simulink model "MMC_phase_discentralized_HAAS_20260927"  (R2024b)
settings: Solver=FixedStepDiscrete  StartTime=t_init_sim  StopTime=sim_time  FixedStep=Ts  RelTol=1e-3
values from neighbouring files (symbols this model uses):
  a = 1    [script_MMC_phase_hackathon_NLM_discentralized_HAAS_20260927.m]
  C1low1_active = 1    [script_MMC_phase_hackathon_NLM_discentralized_HAAS_20260927.m]
  C2low1_active = 1    [script_MMC_phase_hackathon_NLM_discentralized_HAAS_20260927.m]
  C_bus = 4400e-6    (= 0.0044)    [script_MMC_phase_hackathon_NLM_discentralized_HAAS_20260927.m]
  C_M_extra = C_m-twist_high_side_C    [script_MMC_phase_hackathon_NLM_discentralized_HAAS_20260927.m]
  duty_cycle = 1.0    (= 1)    [script_MMC_phase_hackathon_NLM_discentralized_HAAS_20260927.m]
  f0 = 50    [script_MMC_phase_hackathon_NLM_discentralized_HAAS_20260927.m]
  feeder_current_lower_rate_limit = -10    [script_MMC_phase_hackathon_NLM_discentralized_HAAS_20260927.m]    (also in twist_parameters.m = -500)
  feeder_current_tab = [0.328 0.217 0.162 0.132 0.109 0.094 0.083 0.075 0.068 0.062 0.058 0.054 ... (42 elements, 14x3)]    [feeder_current.mat]
  feeder_current_upper_rate_limit = 0.386/(20e-3)    (= 19.3)    [twist_parameters.m]
  is6VExternallySupplied = true    [script_MMC_phase_hackathon_NLM_discentralized_HAAS_20260927.m]
  isFeederJumperOpen = true    [script_MMC_phase_hackathon_NLM_discentralized_HAAS_20260927.m]
  L_arm = 30e-3    (= 0.03)    [script_MMC_phase_hackathon_NLM_discentralized_HAAS_20260927.m]
  m = 1    [script_MMC_phase_hackathon_NLM_discentralized_HAAS_20260927.m]
  N = 5    [script_MMC_phase_hackathon_NLM_discentralized_HAAS_20260927.m]
  power_losses = false    [script_MMC_phase_hackathon_NLM_discentralized_HAAS_20260927.m]
  R = 15    [script_MMC_phase_hackathon_NLM_discentralized_HAAS_20260927.m]
  R_arm = 0.2    [script_MMC_phase_hackathon_NLM_discentralized_HAAS_20260927.m]
  source_V = 0    [script_MMC_phase_hackathon_NLM_discentralized_HAAS_20260927.m]
  Tcom_sample = round(Tcom / Ts)    [script_MMC_phase_hackathon_NLM_discentralized_HAAS_20260927.m]
  time_charge = 0.1    [script_MMC_phase_hackathon_NLM_discentralized_HAAS_20260927.m]
  time_decharge = 1.5    [script_MMC_phase_hackathon_NLM_discentralized_HAAS_20260927.m]
  Ts = 1e-6    (= 1e-06)    [script_MMC_phase_hackathon_NLM_discentralized_HAAS_20260927.m]
  twist_data_acquisition_delay = 50e-9    (= 5e-08)    [script_MMC_phase_hackathon_NLM_discentralized_HAAS_20260927.m]    (also in twist_parameters.m)
  twist_data_sampling_period = 1/twist_freq_data_sampling    (= 5e-05)    [script_MMC_phase_hackathon_NLM_discentralized_HAAS_20260927.m]    (also in twist_parameters.m)
  twist_dead_time = 200e-9    (= 2e-07)    [twist_parameters.m]
  twist_freq_switching = 200e3    (= 200000)    [twist_parameters.m]
  twist_high_side_adc_R = 1/(1/2e6 + 1/2e6 + 1/(330e3+5.6e3))    (= 251272.836178)    [twist_parameters.m]
  twist_high_side_C = 33e-6*4 + 4.7e-6*12    (= 0.0001884)    [twist_parameters.m]
  twist_high_side_feeder_R = 47e3+4.7e3    (= 51700)    [twist_parameters.m]
  twist_high_side_rC = 0.1    [twist_parameters.m]
  twist_low_side_adc_R = 150e3+470    (= 150470)    [twist_parameters.m]
  twist_low_side_C_ceramic = 3*4.7e-6    (= 1.41e-05)    [twist_parameters.m]
  twist_low_side_C_electrolytic = 47e-6    (= 4.7e-05)    [twist_parameters.m]
  twist_low_side_L = 33e-6    (= 3.3e-05)    [twist_parameters.m]
  twist_low_side_rC = 700e-3    (= 0.7)    [twist_parameters.m]
  twist_low_side_rL = 20e-3    (= 0.02)    [twist_parameters.m]
  twist_R_VCC = (tau_VCC/twist_high_side_C  - twist_high_side_rC)/(1-(tau_VCC/twist_high_side_C - twist_high_side_rC)/R_parallel)    (= 1110.74997822)    [twist_parameters.m]
  VDC = 48    [script_MMC_phase_hackathon_NLM_discentralized_HAAS_20260927.m]
undefined symbols (not defined in the file or in its folder): C_SM, feeder_current, gcbh, sps_rtmsupport, twist_low_side_lC
libraries: spsSeriesRLCBranchLib x135, spsTriangleGeneratorLib x60, spsMosfetLib x60, spsCurrentMeasurementLib x43, spsVoltageMeasurementLib x35, spsControlledCurrentSourceLib x30, spsDiodeLib x22, spsIdealSwitchLib x20, spsControlledVoltageSourceLib x1, spsGroundLib x1, spspowerguiLib x1
(part 18 of 22)

== system MMC_phase_discentralized_HAAS_20260927/ /Subsystem/Subsystem1/Hardware M5/HRTimA_1/PWM Generator (2-Level)/Sampling/Unsync Natural/Unsync_NaturalSampling ==
  Uref : Inport  Interpolate=off
  Triangle Generator : spsTriangleGeneratorLib/Triangle Generator  Freq=sps.Fc  Phase=sps.Pc  Ts=Ts
  Uref* : Outport  VectorParamsAs1DForOutWhenUnconnected=off
  Cr : Outport  Port=2  VectorParamsAs1DForOutWhenUnconnected=off
  wires:
  Triangle Generator/1 -> Cr/1
  Uref/1 -> Uref*/1

== system MMC_phase_discentralized_HAAS_20260927/ /Subsystem/Subsystem1/Hardware M5/HRTimA_1/PWM Generator (2-Level)/Sampling/Unsync Symmetrical/Unsync_SymmetricalSampling ==
  Uref : Inport  Interpolate=off
  Triangle Generator : spsTriangleGeneratorLib/Triangle Generator  Freq=sps.Fc  Phase=sps.Pc  Ts=Ts
  Zero-Order Hold : ZeroOrderHold  SampleTime=sps.SampleTimeZOH_SymSampling
  Uref* : Outport  VectorParamsAs1DForOutWhenUnconnected=off
  Cr : Outport  Port=2  VectorParamsAs1DForOutWhenUnconnected=off
  wires:
  Triangle Generator/1 -> Cr/1
  Uref/1 -> Zero-Order Hold/1
  Zero-Order Hold/1 -> Uref*/1

== system MMC_phase_discentralized_HAAS_20260927/ /Subsystem/Subsystem1/Hardware M5/HRTimA_2/PWM Generator (2-Level)/Sampling/Sync Asymmetrical/Sample & Hold ==
  In : Inport
  Enable : EnablePort
  Out : Outport  VectorParamsAs1DForOutWhenUnconnected=off
  wires:
  In/1 -> Out/1

== system MMC_phase_discentralized_HAAS_20260927/ /Subsystem/Subsystem1/Hardware M5/HRTimA_2/PWM Generator (2-Level)/Sampling/Sync Natural/Sync_NaturalSampling ==
  Uref : Inport  Interpolate=off
  wt : Inport  Port=2  Interpolate=off
  Gain1 : Gain  Gain=2/pi  SaturateOnIntegerOverflow=on  OutDataTypeStr=Inherit: Same as input  ParamDataTypeStr=Inherit: Same as input
  Gain4 : Gain  Gain=nF  SaturateOnIntegerOverflow=on  OutDataTypeStr=Inherit: Same as input  ParamDataTypeStr=Inherit: Same as input
  Trigonometric Function : Trigonometry  Operator=asin
  Trigonometric Function3 : Trigonometry
  Uref* : Outport  VectorParamsAs1DForOutWhenUnconnected=off
  Cr : Outport  Port=2  VectorParamsAs1DForOutWhenUnconnected=off
  wires:
  wt/1 -> Gain4/1
  Gain1/1 -> Cr/1
  Trigonometric Function/1 -> Gain1/1
  Trigonometric Function3/1 -> Trigonometric Function/1
  Gain4/1 -> Trigonometric Function3/1
  Uref/1 -> Uref*/1

== system MMC_phase_discentralized_HAAS_20260927/ /Subsystem/Subsystem1/Hardware M5/HRTimA_2/PWM Generator (2-Level)/Sampling/Sync Symmetrical/Sync_SymmetricalSampling ==
  Uref : Inport  Interpolate=off
  wt : Inport  Port=2  Interpolate=off
  Add : Sum
  Constant3 : Constant
  Gain1 : Gain  Gain=2/pi  SaturateOnIntegerOverflow=on  OutDataTypeStr=Inherit: Same as input  ParamDataTypeStr=Inherit: Same as input
  Gain4 : Gain  Gain=nF  SaturateOnIntegerOverflow=on  OutDataTypeStr=Inherit: Same as input  ParamDataTypeStr=Inherit: Same as input
  Hit Crossing : HitCross  HitCrossingOffset=1e-9  HitCrossingDirection=falling
  Sample & Hold : Subsystem
  Trigonometric Function : Trigonometry  Operator=asin
  Trigonometric Function3 : Trigonometry
  Uref* : Outport  VectorParamsAs1DForOutWhenUnconnected=off
  Cr : Outport  Port=2  VectorParamsAs1DForOutWhenUnconnected=off
  wires:
  wt/1 -> Gain4/1
  Gain1/1 -> Cr/1, Add/1
  Trigonometric Function/1 -> Gain1/1
  Trigonometric Function3/1 -> Trigonometric Function/1
  Gain4/1 -> Trigonometric Function3/1
  Add/1 -> Hit Crossing/1
  Constant3/1 -> Add/2
  Hit Crossing/1 -> Sample & Hold/Enable
  Uref/1 -> Sample & Hold/1(In)
  Sample & Hold/1(Out) -> Uref*/1

== system MMC_phase_discentralized_HAAS_20260927/ /Subsystem/Subsystem1/Hardware M5/HRTimA_2/PWM Generator (2-Level)/Sampling/Unsync Asymmetrical/Unsync_AsymmetricalSampling ==
  Uref : Inport  Interpolate=off
  Triangle Generator : spsTriangleGeneratorLib/Triangle Generator  Freq=sps.Fc  Phase=sps.Pc  Ts=Ts
  Zero-Order Hold : ZeroOrderHold  SampleTime=sps.SampleTimeZOH_AsymSampling
  Uref* : Outport  VectorParamsAs1DForOutWhenUnconnected=off
  Cr : Outport  Port=2  VectorParamsAs1DForOutWhenUnconnected=off
  wires:
  Triangle Generator/1 -> Cr/1
  Uref/1 -> Zero-Order Hold/1
  Zero-Order Hold/1 -> Uref*/1

== system MMC_phase_discentralized_HAAS_20260927/ /Subsystem/Subsystem1/Hardware M5/HRTimA_2/PWM Generator (2-Level)/Sampling/Unsync Natural/Unsync_NaturalSampling ==
  Uref : Inport  Interpolate=off
  Triangle Generator : spsTriangleGeneratorLib/Triangle Generator  Freq=sps.Fc  Phase=sps.Pc  Ts=Ts
  Uref* : Outport  VectorParamsAs1DForOutWhenUnconnected=off
  Cr : Outport  Port=2  VectorParamsAs1DForOutWhenUnconnected=off
  wires:
  Triangle Generator/1 -> Cr/1
  Uref/1 -> Uref*/1

== system MMC_phase_discentralized_HAAS_20260927/ /Subsystem/Subsystem1/Hardware M5/HRTimA_2/PWM Generator (2-Level)/Sampling/Unsync Symmetrical/Unsync_SymmetricalSampling ==
  Uref : Inport  Interpolate=off
  Triangle Generator : spsTriangleGeneratorLib/Triangle Generator  Freq=sps.Fc  Phase=sps.Pc  Ts=Ts
  Zero-Order Hold : ZeroOrderHold  SampleTime=sps.SampleTimeZOH_SymSampling
  Uref* : Outport  VectorParamsAs1DForOutWhenUnconnected=off
  Cr : Outport  Port=2  VectorParamsAs1DForOutWhenUnconnected=off
  wires:
  Triangle Generator/1 -> Cr/1
  Uref/1 -> Zero-Order Hold/1
  Zero-Order Hold/1 -> Uref*/1

== system MMC_phase_discentralized_HAAS_20260927/ /Subsystem/Subsystem/Hardware M1/HRTimA_1/PWM Generator (2-Level)/Sampling/Sync Symmetrical/Sync_SymmetricalSampling/Sample & Hold ==
  In : Inport
  Enable : EnablePort
  Out : Outport  VectorParamsAs1DForOutWhenUnconnected=off
  wires:
  In/1 -> Out/1

== system MMC_phase_discentralized_HAAS_20260927/ /Subsystem/Subsystem/Hardware M1/HRTimA_2/PWM Generator (2-Level)/Sampling/Sync Symmetrical/Sync_SymmetricalSampling/Sample & Hold ==
  In : Inport
  Enable : EnablePort
  Out : Outport  VectorParamsAs1DForOutWhenUnconnected=off
  wires:
  In/1 -> Out/1

== system MMC_phase_discentralized_HAAS_20260927/ /Subsystem/Subsystem/Hardware M2/HRTimA_1/PWM Generator (2-Level)/Sampling/Sync Symmetrical/Sync_SymmetricalSampling/Sample & Hold ==
  In : Inport
  Enable : EnablePort
  Out : Outport  VectorParamsAs1DForOutWhenUnconnected=off
  wires:
  In/1 -> Out/1

== system MMC_phase_discentralized_HAAS_20260927/ /Subsystem/Subsystem/Hardware M2/HRTimA_2/PWM Generator (2-Level)/Sampling/Sync Symmetrical/Sync_SymmetricalSampling/Sample & Hold ==
  In : Inport
  Enable : EnablePort
  Out : Outport  VectorParamsAs1DForOutWhenUnconnected=off
  wires:
  In/1 -> Out/1

== system MMC_phase_discentralized_HAAS_20260927/ /Subsystem/Subsystem/Hardware M3/HRTimA_1/PWM Generator (2-Level)/Sampling/Sync Symmetrical/Sync_SymmetricalSampling/Sample & Hold ==
  In : Inport
  Enable : EnablePort
  Out : Outport  VectorParamsAs1DForOutWhenUnconnected=off
  wires:
  In/1 -> Out/1

== system MMC_phase_discentralized_HAAS_20260927/ /Subsystem/Subsystem/Hardware M3/HRTimA_2/PWM Generator (2-Level)/Sampling/Sync Symmetrical/Sync_SymmetricalSampling/Sample & Hold ==
  In : Inport
  Enable : EnablePort
  Out : Outport  VectorParamsAs1DForOutWhenUnconnected=off
  wires:
  In/1 -> Out/1

== system MMC_phase_discentralized_HAAS_20260927/ /Subsystem/Subsystem/Hardware M4/HRTimA_1/PWM Generator (2-Level)/Sampling/Sync Symmetrical/Sync_SymmetricalSampling/Sample & Hold ==
  In : Inport
  Enable : EnablePort
  Out : Outport  VectorParamsAs1DForOutWhenUnconnected=off
  wires:
  In/1 -> Out/1

== system MMC_phase_discentralized_HAAS_20260927/ /Subsystem/Subsystem/Hardware M4/HRTimA_2/PWM Generator (2-Level)/Sampling/Sync Symmetrical/Sync_SymmetricalSampling/Sample & Hold ==
  In : Inport
  Enable : EnablePort
  Out : Outport  VectorParamsAs1DForOutWhenUnconnected=off
  wires:
  In/1 -> Out/1

== system MMC_phase_discentralized_HAAS_20260927/ /Subsystem/Subsystem/Hardware M5/HRTimA_1/PWM Generator (2-Level)/Sampling/Sync Symmetrical/Sync_SymmetricalSampling/Sample & Hold ==
  In : Inport
  Enable : EnablePort
  Out : Outport  VectorParamsAs1DForOutWhenUnconnected=off
  wires:
  In/1 -> Out/1

== system MMC_phase_discentralized_HAAS_20260927/ /Subsystem/Subsystem/Hardware M5/HRTimA_2/PWM Generator (2-Level)/Sampling/Sync Symmetrical/Sync_SymmetricalSampling/Sample & Hold ==
  In : Inport
  Enable : EnablePort
  Out : Outport  VectorParamsAs1DForOutWhenUnconnected=off
  wires:
  In/1 -> Out/1

== system MMC_phase_discentralized_HAAS_20260927/ /Subsystem/Subsystem1/Hardware M1/HRTimA_1/PWM Generator (2-Level)/Sampling/Sync Symmetrical/Sync_SymmetricalSampling/Sample & Hold ==
  In : Inport
  Enable : EnablePort
  Out : Outport  VectorParamsAs1DForOutWhenUnconnected=off
  wires:
  In/1 -> Out/1

== system MMC_phase_discentralized_HAAS_20260927/ /Subsystem/Subsystem1/Hardware M1/HRTimA_2/PWM Generator (2-Level)/Sampling/Sync Symmetrical/Sync_SymmetricalSampling/Sample & Hold ==
  In : Inport
  Enable : EnablePort
  Out : Outport  VectorParamsAs1DForOutWhenUnconnected=off
  wires:
  In/1 -> Out/1

== system MMC_phase_discentralized_HAAS_20260927/ /Subsystem/Subsystem1/Hardware M2/HRTimA_1/PWM Generator (2-Level)/Sampling/Sync Symmetrical/Sync_SymmetricalSampling/Sample & Hold ==
  In : Inport
  Enable : EnablePort
  Out : Outport  VectorParamsAs1DForOutWhenUnconnected=off
  wires:
  In/1 -> Out/1

== system MMC_phase_discentralized_HAAS_20260927/ /Subsystem/Subsystem1/Hardware M2/HRTimA_2/PWM Generator (2-Level)/Sampling/Sync Symmetrical/Sync_SymmetricalSampling/Sample & Hold ==
  In : Inport
  Enable : EnablePort
  Out : Outport  VectorParamsAs1DForOutWhenUnconnected=off
  wires:
  In/1 -> Out/1

== system MMC_phase_discentralized_HAAS_20260927/ /Subsystem/Subsystem1/Hardware M3/HRTimA_1/PWM Generator (2-Level)/Sampling/Sync Symmetrical/Sync_SymmetricalSampling/Sample & Hold ==
  In : Inport
  Enable : EnablePort
  Out : Outport  VectorParamsAs1DForOutWhenUnconnected=off
  wires:
  In/1 -> Out/1

== system MMC_phase_discentralized_HAAS_20260927/ /Subsystem/Subsystem1/Hardware M3/HRTimA_2/PWM Generator (2-Level)/Sampling/Sync Symmetrical/Sync_SymmetricalSampling/Sample & Hold ==
  In : Inport
  Enable : EnablePort
  Out : Outport  VectorParamsAs1DForOutWhenUnconnected=off
  wires:
  In/1 -> Out/1

== system MMC_phase_discentralized_HAAS_20260927/ /Subsystem/Subsystem1/Hardware M4/HRTimA_1/PWM Generator (2-Level)/Sampling/Sync Symmetrical/Sync_SymmetricalSampling/Sample & Hold ==
  In : Inport
  Enable : EnablePort
  Out : Outport  VectorParamsAs1DForOutWhenUnconnected=off
  wires:
  In/1 -> Out/1

== system MMC_phase_discentralized_HAAS_20260927/ /Subsystem/Subsystem1/Hardware M4/HRTimA_2/PWM Generator (2-Level)/Sampling/Sync Symmetrical/Sync_SymmetricalSampling/Sample & Hold ==
  In : Inport
  Enable : EnablePort
  Out : Outport  VectorParamsAs1DForOutWhenUnconnected=off
  wires:
  In/1 -> Out/1

== system MMC_phase_discentralized_HAAS_20260927/ /Subsystem/Subsystem1/Hardware M5/HRTimA_1/PWM Generator (2-Level)/Sampling/Sync Symmetrical/Sync_SymmetricalSampling/Sample & Hold ==
  In : Inport
  Enable : EnablePort
  Out : Outport  VectorParamsAs1DForOutWhenUnconnected=off
  wires:
  In/1 -> Out/1

== system MMC_phase_discentralized_HAAS_20260927/ /Subsystem/Subsystem1/Hardware M5/HRTimA_2/PWM Generator (2-Level)/Sampling/Sync Symmetrical/Sync_SymmetricalSampling/Sample & Hold ==
  In : Inport
  Enable : EnablePort
  Out : Outport  VectorParamsAs1DForOutWhenUnconnected=off
  wires:
  In/1 -> Out/1

== matlab function MMC_phase_discentralized_HAAS_20260927/ /Communication_subsystem/Upper_arm/M2_Comm/Snapshot ==
  data: rx_signal input uint64; local_frame_snapshot input; rx_variables output single; sync input; round_done input
function rx_variables = Snapshot_block(rx_signal, local_frame_snapshot, sync, round_done)
%#codegen
%
% Snapshot block SSAF.
%
% Comportement voulu :
%   - pendant le round, les trames reçues mettent à jour working_bank ;
%   - local_frame_snapshot met à jour la donnée locale ;
%   - au front montant de sync, published_snapshot = working_bank ;
%   - le contrôle lit published_snapshot pendant la période de contrôle.
%
% round_done est conservé dans l'interface pour debug, mais la publication
% du snapshot se fait sur le front montant de sync.

% =========================
% Paramètres
% =========================
VC_LSB = single(0.1);
I_LSB  = single(0.1);

% =========================
% Etats persistants
% =========================
persistent working_bank
persistent published_snapshot
persistent sync_z
persistent last_rx_word
persistent last_rx_valid

if isempty(working_bank)
    working_bank = zeros(12, 1, 'single');
end

if isempty(published_snapshot)
    published_snapshot = zeros(12, 1, 'single');
end

if isempty(sync_z)
    sync_z = false;
end

if isempty(last_rx_word)
    last_rx_word = uint64(0);
end

if isempty(last_rx_valid)
    last_rx_valid = false;
end

% =========================
% Détection fronts sync
% =========================
sync_bool = sync ~= 0;
rise_sync = sync_bool && ~sync_z;

% =========================================================
% 1) Publication du snapshot au front montant
%
% Important :
%   published_snapshot est mis à jour AVANT la sortie.
%   Il contient les données reçues jusqu'au pas précédent.
%   Une trame qui arrive exactement au même pas que rise_sync est traitée
%   plus bas et sera donc visible au prochain front montant.
% =========================================================
if rise_sync
    published_snapshot = working_bank;
end

% =========================================================
% 2) Sortie enregistrée
%
% rx_variables ne dépend pas directement de rx_signal ou
% local_frame_snapshot au même pas de simulation.
% Cela évite une boucle algébrique avec le CVB.
% =========================================================
rx_variables = published_snapshot;

% Petit usage de round_done pour éviter qu'il soit complètement inutilisé.
% Il ne déclenche pas la publication.
if round_done ~= 0
    published_snapshot = published_snapshot;
end

% =========================
% 3) Mise à jour avec la trame locale
%
% local_frame_snapshot est émis seulement quand un nouveau round démarre.
% =========================
local_word = uint64(local_frame_snapshot(1));

[local_valid, local_current_present, local_id, local_vc, local_iarm] = ...
    unpack_frame(local_word, VC_LSB, I_LSB);

if local_valid
    working_bank = update_bank_from_frame(working_bank, ...
                                          local_valid, ...
                                          local_current_present, ...
                                          local_id, ...
                                          local_vc, ...
                                          local_iarm);
end

% =========================
% 4) Mise à jour avec la trame reçue depuis l'anneau
% =========================
rx_word = uint64(rx_signal(1));

[rx_valid, rx_current_present, rx_id, rx_vc, rx_iarm] = ...
    unpack_frame(rx_word, VC_LSB, I_LSB);

new_rx = rx_valid && ((rx_word ~= last_rx_word) || ~last_rx_valid);

if new_rx
    working_bank = update_bank_from_frame(working_bank, ...
                                          rx_valid, ...
                                          rx_current_present, ...
                                          rx_id, ...
                                          rx_vc, ...
                                          rx_iarm);
end

% =========================
% Mise à jour mémoires
% =========================
sync_z = sync_bool;

last_rx_word  = rx_word;
last_rx_valid = rx_valid;


% =========================================================
% UPDATE BANK FROM FRAME
% =========================================================
function bank_out = update_bank_from_frame(bank_in, valid, current_present, id, vc, iarm)
%#codegen

    bank_out = bank_in;

    if ~valid
        return;
    end

    % Upper arm : ID 1 à 5
    if id >= uint8(1) && id <= uint8(5)

        idx = double(id);          % ID 1 -> bank(1), ..., ID 5 -> bank(5)
        bank_out(idx) = single(vc);

        % Seul M1 transporte I_u
        if id == uint8(1) && current_present
            bank_out(6) = single(iarm);
        end

    % Lower arm : ID 6 à 10
    elseif id >= uint8(6) && id <= uint8(10)

        idx = 6 + double(id - uint8(5));  % ID 6 -> bank(7), ..., ID 10 -> bank(11)
        bank_out(idx) = single(vc);

        % Seul M6 transporte I_l
        if id == uint8(6) && current_present
            bank_out(12) = single(iarm);
        end
    end
end


% =========================================================
% UNPACK FRAME
%
% Format uint64:
%   bit 41      : valid
%   bit 40      : current_present
%   bits 39..32 : node_id
%   bits 31..16 : Vc local, uint16
%   bits 15..0  : I arm, int16 encodé en complément à deux
% =========================================================
function [valid, current_present, id, vc, iarm] = unpack_frame(frame, vc_lsb, i_lsb)
%#codegen

    frame_scalar = uint64(frame(1));

    valid = bitand(bitshift(frame_scalar, -41), uint64(1)) ~= uint64(0);
    current_present = bitand(bitshift(frame_scalar, -40), uint64(1)) ~= uint64(0);

    id = uint8(bitand(bitshift(frame_scalar, -32), uint64(255)));

    vc_q = uint16(bitand(bitshift(frame_scalar, -16), uint64(65535)));
    vc = single(double(vc_q) * double(vc_lsb));

    i_u16 = uint16(bitand(frame_scalar, uint64(65535)));

    if i_u16 >= uint16(32768)
        i_q_double = double(i_u16) - 65536;
    else
        i_q_double = double(i_u16);
    end

    iarm = single(i_q_double * double(i_lsb));
end

end

== matlab function MMC_phase_discentralized_HAAS_20260927/ /Sinus Modulation + Sorting Algorithm/M2 MCU/Sorting/Tri2 ==
  data: ordre output; Vcp input; i input; sens output
function [ordre,sens] = fcn(Vcp, i)

[~, ordre] = sort(Vcp);

if i >= 0 
    sens = 1;
else 
    sens = 0;
end

% ordre = [1,2,3,4,5]';
% sens = 1;

== matlab function MMC_phase_discentralized_HAAS_20260927/ /Sinus Modulation + Sorting Algorithm/M3 MCU/CVB ==
  data: ordre input; y output; sens input; N_on input; duty_cycle input; M_number input
function y = fcn(ordre,sens,N_on,duty_cycle,M_number)

N_m = length(ordre);
Gp = zeros(1,2);
Ap0=ordre;
kp = find(ordre == M_number);
%% Positive direction (sens = 1)
if sens==1         % ON the capacitors least charged
    
    if kp <= N_on
        %K1 = 1 ; K2 = 0
        Gp(1)=duty_cycle;
        Gp(2)=-0.01;
    else
        %K1 = 0 ; K2 = 1
        Gp(1)=-0.01;
        Gp(2)=duty_cycle;
    end

else            % ON the capacitors most charged
    
    if kp > N_m - N_on
        %K1 = 1 ; K2 = 0
        Gp(1)=duty_cycle;
        Gp(2)=-0.01;
        
    else
        %K1 = 0 ; K2 = 1
        Gp(1)=-0.01;
        Gp(2)=duty_cycle;
    end

end
y=Gp';

== matlab function MMC_phase_discentralized_HAAS_20260927/ /Sinus Modulation + Sorting Algorithm/M3 MCU/Sorting/Tri2 ==
  data: ordre output; Vcp input; i input; sens output
function [ordre,sens] = fcn(Vcp, i)

[~, ordre] = sort(Vcp);

if i >= 0 
    sens = 1;
else 
    sens = 0;
end

% ordre = [1,2,3,4,5]';
% sens = 1;

== matlab function MMC_phase_discentralized_HAAS_20260927/ /Communication_subsystem/Communication architecture/MATLAB Function ==
  data: M1_TX_Signal input; bus_signal output; M2_TX_Signal input; M3_TX_Signal input; collision output; M4_TX_Signal input; M5_TX_Signal input; M6_TX_Signal input; M7_TX_Signal input; M8_TX_Signal input; M9_TX_Signal input; M10_TX_Signal input
function [bus_signal, collision] = Bus_Arbitration( ...
    M1_TX_Signal, M2_TX_Signal, M3_TX_Signal, M4_TX_Signal, M5_TX_Signal, ...
    M6_TX_Signal, M7_TX_Signal, M8_TX_Signal, M9_TX_Signal, M10_TX_Signal)
%#codegen

signals = repmat(uint64(0), 10, 1);

signals(1)  = M1_TX_Signal;
signals(2)  = M2_TX_Signal;
signals(3)  = M3_TX_Signal;
signals(4)  = M4_TX_Signal;
signals(5)  = M5_TX_Signal;
signals(6)  = M6_TX_Signal;
signals(7)  = M7_TX_Signal;
signals(8)  = M8_TX_Signal;
signals(9)  = M9_TX_Signal;
signals(10) = M10_TX_Signal;

count_active = uint8(0);
last_signal  = uint64(0);

for k = 1:10
    if signals(k) ~= uint64(0)
        count_active = count_active + 1;
        last_signal = signals(k);
    end
end

if count_active == uint8(0)
    bus_signal = uint64(0);
    collision = false;
elseif count_active == uint8(1)
    bus_signal = last_signal;
    collision = false;
else
    % Collision : deux modules ou plus emettent en meme temps
    bus_signal = uint64(0);
    collision = true;
end

end

== matlab function MMC_phase_discentralized_HAAS_20260927/ /Sinus Modulation + Sorting Algorithm/M4 MCU/CVB ==
  data: ordre input; y output; sens input; N_on input; duty_cycle input; M_number input
function y = fcn(ordre,sens,N_on,duty_cycle,M_number)

N_m = length(ordre);
Gp = zeros(1,2);
Ap0=ordre;
kp = find(ordre == M_number);
%% Positive direction (sens = 1)
if sens==1         % ON the capacitors least charged
    
    if kp <= N_on
        %K1 = 1 ; K2 = 0
        Gp(1)=duty_cycle;
        Gp(2)=-0.01;
    else
        %K1 = 0 ; K2 = 1
        Gp(1)=-0.01;
        Gp(2)=duty_cycle;
    end

else            % ON the capacitors most charged
    
    if kp > N_m - N_on
        %K1 = 1 ; K2 = 0
        Gp(1)=duty_cycle;
        Gp(2)=-0.01;
        
    else
        %K1 = 0 ; K2 = 1
        Gp(1)=-0.01;
        Gp(2)=duty_cycle;
    end

end
y=Gp';

== matlab function MMC_phase_discentralized_HAAS_20260927/ /Sinus Modulation + Sorting Algorithm/M4 MCU/Sorting/Tri2 ==
  data: ordre output; Vcp input; i input; sens output
function [ordre,sens] = fcn(Vcp, i)

[~, ordre] = sort(Vcp);

if i >= 0 
    sens = 1;
else 
    sens = 0;
end

% ordre = [1,2,3,4,5]';
% sens = 1;

== matlab function MMC_phase_discentralized_HAAS_20260927/ /Sinus Modulation + Sorting Algorithm/M5 MCU/CVB ==
  data: ordre input; y output; sens input; N_on input; duty_cycle input; M_number input
function y = fcn(ordre,sens,N_on,duty_cycle,M_number)

N_m = length(ordre);
Gp = zeros(1,2);
Ap0=ordre;
kp = find(ordre == M_number);
%% Positive direction (sens = 1)
if sens==1         % ON the capacitors least charged
    
    if kp <= N_on
        %K1 = 1 ; K2 = 0
        Gp(1)=duty_cycle;
        Gp(2)=-0.01;
    else
        %K1 = 0 ; K2 = 1
        Gp(1)=-0.01;
        Gp(2)=duty_cycle;
    end

else            % ON the capacitors most charged
    
    if kp > N_m - N_on
        %K1 = 1 ; K2 = 0
        Gp(1)=duty_cycle;
        Gp(2)=-0.01;
        
    else
        %K1 = 0 ; K2 = 1
        Gp(1)=-0.01;
        Gp(2)=duty_cycle;
    end

end
y=Gp';

== matlab function MMC_phase_discentralized_HAAS_20260927/ /Sinus Modulation + Sorting Algorithm/M5 MCU/Sorting/Tri2 ==
  data: ordre output; Vcp input; i input; sens output
function [ordre,sens] = fcn(Vcp, i)

[~, ordre] = sort(Vcp);

if i >= 0 
    sens = 1;
else 
    sens = 0;
end

% ordre = [1,2,3,4,5]';
% sens = 1;

== matlab function MMC_phase_discentralized_HAAS_20260927/ /Sinus Modulation + Sorting Algorithm/M6 MCU/CVB ==
  data: ordre input; y output; sens input; N_on input; duty_cycle input; M_number input
function y = fcn(ordre,sens,N_on,duty_cycle,M_number)

N_m = length(ordre);
Gp = zeros(1,2);
Ap0=ordre;
kp = find(ordre == M_number);
%% Positive direction (sens = 1)
if sens==1         % ON the capacitors least charged
    
    if kp <= N_on
        %K1 = 1 ; K2 = 0
        Gp(1)=duty_cycle;
        Gp(2)=-0.01;
    else
        %K1 = 0 ; K2 = 1
        Gp(1)=-0.01;
        Gp(2)=duty_cycle;
    end

else            % ON the capacitors most charged
    
    if kp > N_m - N_on
        %K1 = 1 ; K2 = 0
        Gp(1)=duty_cycle;
        Gp(2)=-0.01;
        
    else
        %K1 = 0 ; K2 = 1
        Gp(1)=-0.01;
        Gp(2)=duty_cycle;
    end

end
y=Gp';

== matlab function MMC_phase_discentralized_HAAS_20260927/ /Sinus Modulation + Sorting Algorithm/M6 MCU/Sorting/Tri2 ==
  data: ordre output; Vcp input; i input; sens output
function [ordre,sens] = fcn(Vcp, i)

[~, ordre] = sort(Vcp);

if i >= 0 
    sens = 1;
else 
    sens = 0;
end

% ordre = [1,2,3,4,5]';
% sens = 1;

== matlab function MMC_phase_discentralized_HAAS_20260927/ /Subsystem/Subsystem1/Hardware M1/Feeder block/MATLAB Function ==
  data: i_feeder input; vC input; isfeederdisabled input; active_1 input; y output; Q_VCC output
function [y,Q_VCC]  = feeder_characteristics(i_feeder,vC,isfeederdisabled,active_1)

if(isfeederdisabled == 1)
    if(vC>=9.7)
        y = 11.2e-3;
        Q_VCC = 0;
    elseif(vC>=8.9 && vC < 9.7)
        if(active_1 == true)
            y = 11.2e-3;
            Q_VCC = 0;
        else
            y = 0;
            Q_VCC = 1;
        end
    else
        y = 0;
        Q_VCC = 1;
    end
else
    if(vC>=9.7)
        y = i_feeder;
        Q_VCC = 0;
    elseif(vC>=8.9 && vC < 9.7)
        if(active_1 == true)
            y = i_feeder;
            Q_VCC = 0;
        else
            y = 0;
            Q_VCC = 1;
        end
    else
        y = 0;
        Q_VCC = 1;
    end
end

== matlab function MMC_phase_discentralized_HAAS_20260927/ /Sinus Modulation + Sorting Algorithm/M7 MCU/CVB ==
  data: ordre input; y output; sens input; N_on input; duty_cycle input; M_number input
function y = fcn(ordre,sens,N_on,duty_cycle,M_number)

N_m = length(ordre);
Gp = zeros(1,2);
Ap0=ordre;
kp = find(ordre == M_number);
%% Positive direction (sens = 1)
if sens==1         % ON the capacitors least charged
    
    if kp <= N_on
        %K1 = 1 ; K2 = 0
        Gp(1)=duty_cycle;
        Gp(2)=-0.01;
    else
        %K1 = 0 ; K2 = 1
        Gp(1)=-0.01;
        Gp(2)=duty_cycle;
    end

else            % ON the capacitors most charged
    
    if kp > N_m - N_on
        %K1 = 1 ; K2 = 0
        Gp(1)=duty_cycle;
        Gp(2)=-0.01;
        
    else
        %K1 = 0 ; K2 = 1
        Gp(1)=-0.01;
        Gp(2)=duty_cycle;
    end

end
y=Gp';

== matlab function MMC_phase_discentralized_HAAS_20260927/ /Sinus Modulation + Sorting Algorithm/M7 MCU/Sorting/Tri2 ==
  data: ordre output; Vcp input; i input; sens output
function [ordre,sens] = fcn(Vcp, i)

[~, ordre] = sort(Vcp);

if i >= 0 
    sens = 1;
else 
    sens = 0;
end

% ordre = [1,2,3,4,5]';
% sens = 1;

== matlab function MMC_phase_discentralized_HAAS_20260927/ /Sinus Modulation + Sorting Algorithm/M8 MCU/CVB ==
  data: ordre input; y output; sens input; N_on input; duty_cycle input; M_number input
function y = fcn(ordre,sens,N_on,duty_cycle,M_number)

N_m = length(ordre);
Gp = zeros(1,2);
Ap0=ordre;
kp = find(ordre == M_number);
%% Positive direction (sens = 1)
if sens==1         % ON the capacitors least charged
    
    if kp <= N_on
        %K1 = 1 ; K2 = 0
        Gp(1)=duty_cycle;
        Gp(2)=-0.01;
    else
        %K1 = 0 ; K2 = 1
        Gp(1)=-0.01;
        Gp(2)=duty_cycle;
    end

else            % ON the capacitors most charged
    
    if kp > N_m - N_on
        %K1 = 1 ; K2 = 0
        Gp(1)=duty_cycle;
        Gp(2)=-0.01;
        
    else
        %K1 = 0 ; K2 = 1
        Gp(1)=-0.01;
        Gp(2)=duty_cycle;
    end

end
y=Gp';

== matlab function MMC_phase_discentralized_HAAS_20260927/ /Sinus Modulation + Sorting Algorithm/M8 MCU/Sorting/Tri2 ==
  data: ordre output; Vcp input; i input; sens output
function [ordre,sens] = fcn(Vcp, i)

[~, ordre] = sort(Vcp);

if i >= 0 
    sens = 1;
else 
    sens = 0;
end

% ordre = [1,2,3,4,5]';
% sens = 1;

== matlab function MMC_phase_discentralized_HAAS_20260927/ /Sinus Modulation + Sorting Algorithm/M9 MCU/CVB ==
  data: ordre input; y output; sens input; N_on input; duty_cycle input; M_number input
function y = fcn(ordre,sens,N_on,duty_cycle,M_number)

N_m = length(ordre);
Gp = zeros(1,2);
Ap0=ordre;
kp = find(ordre == M_number);
%% Positive direction (sens = 1)
if sens==1         % ON the capacitors least charged
    
    if kp <= N_on
        %K1 = 1 ; K2 = 0
        Gp(1)=duty_cycle;
        Gp(2)=-0.01;
    else
        %K1 = 0 ; K2 = 1
        Gp(1)=-0.01;
        Gp(2)=duty_cycle;
    end

else            % ON the capacitors most charged
    
    if kp > N_m - N_on
        %K1 = 1 ; K2 = 0
        Gp(1)=duty_cycle;
        Gp(2)=-0.01;
        
    else
        %K1 = 0 ; K2 = 1
        Gp(1)=-0.01;
        Gp(2)=duty_cycle;
    end

end
y=Gp';

== matlab function MMC_phase_discentralized_HAAS_20260927/ /Sinus Modulation + Sorting Algorithm/M9 MCU/Sorting/Tri2 ==
  data: ordre output; Vcp input; i input; sens output
function [ordre,sens] = fcn(Vcp, i)

[~, ordre] = sort(Vcp);

if i >= 0 
    sens = 1;
else 
    sens = 0;
end

% ordre = [1,2,3,4,5]';
% sens = 1;

== matlab function MMC_phase_discentralized_HAAS_20260927/ /Sinus Modulation + Sorting Algorithm/M10 MCU/CVB ==
  data: ordre input; y output; sens input; N_on input; duty_cycle input; M_number input
function y = fcn(ordre,sens,N_on,duty_cycle,M_number)

N_m = length(ordre);
Gp = zeros(1,2);
Ap0=ordre;
kp = find(ordre == M_number);
%% Positive direction (sens = 1)
if sens==1         % ON the capacitors least charged
    
    if kp <= N_on
        %K1 = 1 ; K2 = 0
        Gp(1)=duty_cycle;
        Gp(2)=-0.01;
    else
        %K1 = 0 ; K2 = 1
        Gp(1)=-0.01;
        Gp(2)=duty_cycle;
    end

else            % ON the capacitors most charged
    
    if kp > N_m - N_on
        %K1 = 1 ; K2 = 0
        Gp(1)=duty_cycle;
        Gp(2)=-0.01;
        
    else
        %K1 = 0 ; K2 = 1
        Gp(1)=-0.01;
        Gp(2)=duty_cycle;
    end

end
y=Gp';

== matlab function MMC_phase_discentralized_HAAS_20260927/ /Sinus Modulation + Sorting Algorithm/M10 MCU/Sorting/Tri2 ==
  data: ordre output; Vcp input; i input; sens output
function [ordre,sens] = fcn(Vcp, i)

[~, ordre] = sort(Vcp);

if i >= 0 
    sens = 1;
else 
    sens = 0;
end

% ordre = [1,2,3,4,5]';
% sens = 1;

== matlab function MMC_phase_discentralized_HAAS_20260927/ /Sinus Modulation + Sorting Algorithm/M1 MCU/CVB ==
  data: ordre input; y output; sens input; N_on input; duty_cycle input; M_number input
function y = fcn(ordre,sens,N_on,duty_cycle,M_number)

N_m = length(ordre);
Gp = zeros(1,2);
Ap0=ordre;
kp = find(ordre == M_number);
%% Positive direction (sens = 1)
if sens==1         % ON the capacitors least charged
    
    if kp <= N_on
        %K1 = 1 ; K2 = 0
        Gp(1)=duty_cycle;
        Gp(2)=-0.01;
    else
        %K1 = 0 ; K2 = 1
        Gp(1)=-0.01;
        Gp(2)=duty_cycle;
    end

else            % ON the capacitors most charged
    
    if kp > N_m - N_on
        %K1 = 1 ; K2 = 0
        Gp(1)=duty_cycle;
        Gp(2)=-0.01;
        
    else
        %K1 = 0 ; K2 = 1
        Gp(1)=-0.01;
        Gp(2)=duty_cycle;
    end

end
y=Gp';

== matlab function MMC_phase_discentralized_HAAS_20260927/ /Sinus Modulation + Sorting Algorithm/M1 MCU/Sorting/Tri2 ==
  data: ordre output; Vcp input; i input; sens output
function [ordre,sens] = fcn(Vcp, i)

[~, ordre] = sort(Vcp);

if i >= 0 
    sens = 1;
else 
    sens = 0;
end

% ordre = [1,2,3,4,5]';
% sens = 1;

== matlab function MMC_phase_discentralized_HAAS_20260927/ /Communication_subsystem/Upper_arm/M2_Comm/TxFormatter ==
  data: tx_variables input single; tx_data output uint64; sync input; rx_signal input uint64; tx_fire output; tx_busy output; node_id input; round_done output; rx_count_dbg output; rx_id_dbg output; overrun output; local_frame_snapshot output
function [tx_data, tx_fire, tx_busy, round_done, rx_count_dbg, rx_id_dbg, overrun, local_frame_snapshot] = ...
    Transmitter_block_SSAF(tx_variables, sync, rx_signal, node_id)
%#codegen
%
% SSAF transmitter sans délai interne.
%
% Le délai Tcom est EXTERNE :
%
%   tx_data -> Discrete Delay(Kcom) -> TX_signal -> RX_signal du voisin
%
% Règle temporelle :
%   - front montant de sync  : publication du snapshot dans Snapshot_block
%   - front descendant sync  : demande de nouveau round
%   - le nouveau round démarre seulement si le round précédent est fini
%
% Si un front descendant arrive alors que le round précédent est actif,
% le front est ignoré. Aucun round ne démarre automatiquement à la fin
% du round courant. Le démarrage suivant attendra le prochain front
% descendant de sync.

% =========================
% Paramètres
% =========================
N_NODES = uint8(10);

VC_LSB = single(0.1);   % 0.1 V / bit
I_LSB  = single(0.1);   % 0.1 A / bit

id_local = uint8(node_id);

% =========================
% Etats internes
% =========================
persistent sync_z
persistent active
persistent rx_count
persistent rx_seen_mask
persistent last_rx_word
persistent last_rx_valid

if isempty(sync_z)
    sync_z        = false;
    active        = false;
    rx_count      = uint8(0);
    rx_seen_mask  = uint32(0);
    last_rx_word  = uint64(0);
    last_rx_valid = false;
end

% =========================
% Valeurs par défaut
% =========================
tx_data              = uint64(0);
tx_fire              = false;
round_done           = false;
overrun              = false;
rx_id_dbg            = uint8(0);
rx_count_dbg         = rx_count;
local_frame_snapshot = uint64(0);

% =========================
% Détection des fronts sync
% =========================
sync_bool = sync ~= 0;

% Front montant : sync 0 -> 1
rise_sync = sync_bool && ~sync_z;

% Front descendant : sync 1 -> 0
fall_sync = (~sync_bool) && sync_z;

% =========================
% Décodage RX
% =========================
rx_word  = uint64(rx_signal(1));
rx_valid = frame_is_valid(rx_word);

% Nouvelle trame si :
%   - trame valide ;
%   - pas simplement la même valeur maintenue plusieurs pas.
new_rx = rx_valid && ((rx_word ~= last_rx_word) || ~last_rx_valid);

% =========================================================
% 1) Traitement RX / relais du round courant
% =========================================================
if active && new_rx

    rx_id = get_frame_id(rx_word);
    rx_id_dbg = rx_id;

    % On relaie uniquement les trames appartenant à d'autres modules.
    % La trame locale, si elle revient, est ignorée.
    if rx_id >= uint8(1) && rx_id <= N_NODES && rx_id ~= id_local

        bit_id = bitshift(uint32(1), int32(rx_id) - int32(1));
        already_seen = bitand(rx_seen_mask, bit_id) ~= uint32(0);

        if ~already_seen
            rx_seen_mask = bitor(rx_seen_mask, bit_id);

            if rx_count < (N_NODES - uint8(1))
                rx_count = rx_count + uint8(1);
            end
        end

        % Pour N = 10 :
        %   rx_count = 1..8 -> relais
        %   rx_count = 9    -> dernière trame reçue, pas de relais
        if (~already_seen) && rx_count < (N_NODES - uint8(1))

            tx_data = rx_word;
            tx_fire = true;

        else

            tx_data = uint64(0);
            tx_fire = false;
        end

        % Fin du round après réception des N-1 trames distantes.
        if rx_count >= (N_NODES - uint8(1))
            active = false;
            round_done = true;
        end

    else
        % Trame locale revenue ou ID invalide : on ne relaie pas.
        tx_data = uint64(0);
        tx_fire = false;
    end
end

% =========================================================
% 2) Demande de nouveau round au front descendant
%
% Le front descendant démarre un round uniquement si le round courant
% est terminé.
% =========================================================
if fall_sync

    if active

        % Le round précédent n'est pas fini.
        % On ne démarre PAS de nouveau round.
        % Ce front de sync est donc manqué.
        overrun = true;

    else

        % Round libre : démarrage immédiat du nouveau round.
        active       = true;
        rx_count     = uint8(0);
        rx_seen_mask = uint32(0);

        last_rx_word  = uint64(0);
        last_rx_valid = false;

        local_frame = build_local_frame(tx_variables, id_local, VC_LSB, I_LSB);

        % Voie communication vers le voisin, avec délai externe z^-Kcom
        tx_data = local_frame;
        tx_fire = frame_is_valid(local_frame);

        % Voie locale vers Snapshot_block, sans délai de communication
        local_frame_snapshot = local_frame;

        % Debug : ID transmis localement
        rx_id_dbg = id_local;
    end
end

% =========================
% 3) Etat busy
% =========================
% Ici tx_busy signifie : round SSAF actif.
tx_busy = active;

% Debug
rx_count_dbg = rx_count;

% Mise à jour des mémoires
sync_z        = sync_bool;
last_rx_word  = rx_word;
last_rx_valid = rx_valid;


% =========================================================
% BUILD LOCAL FRAME
% =========================================================
function frame = build_local_frame(tx_variables, id_local, vc_lsb, i_lsb)
%#codegen

    u = single(tx_variables(:));

    % Indice local dans le bras
    if id_local >= uint8(1) && id_local <= uint8(5)
        local_idx = double(id_local);             % upper: 1..5
    elseif id_local >= uint8(6) && id_local <= uint8(10)
        local_idx = double(id_local - uint8(5));  % lower: 1..5
    else
        local_idx = 1;
    end

    % Tension de condensateur locale
    vc_local = single(u(local_idx));

    % Courant de bras transmis seulement par M1 et M6
    current_present = false;
    i_arm = single(0);

    if (id_local == uint8(1)) || (id_local == uint8(6))
        current_present = true;
        i_arm = single(u(end));
    end

    vc_local = single(vc_local(1));
    i_arm    = single(i_arm(1));

    frame_tmp = pack_frame(true, current_present, id_local, ...
                           vc_local, i_arm, vc_lsb, i_lsb);

    frame = uint64(frame_tmp(1));
end


% =========================================================
% FRAME VALID
% =========================================================
function ok = frame_is_valid(frame)
%#codegen

    frame_scalar = uint64(frame(1));
    ok = bitand(bitshift(frame_scalar, -41), uint64(1)) ~= uint64(0);
end


% =========================================================
% GET FRAME ID
% =========================================================
function id = get_frame_id(frame)
%#codegen

    frame_scalar = uint64(frame(1));
    valid = bitand(bitshift(frame_scalar, -41), uint64(1)) ~= uint64(0);

    if valid
        id = uint8(bitand(bitshift(frame_scalar, -32), uint64(255)));
    else
        id = uint8(0);
    end
end


% =========================================================
% PACK FRAME
%
% Format uint64:
%   bit 41      : valid
%   bit 40      : current_present
%   bits 39..32 : node_id
%   bits 31..16 : Vc local, uint16
%   bits 15..0  : I arm, int16 encodé en complément à deux
% =========================================================
function frame = pack_frame(valid, current_present, id, vc, iarm, vc_lsb, i_lsb)
%#codegen

    vc_scalar   = single(vc(1));
    iarm_scalar = single(iarm(1));
    id_scalar   = uint8(id(1));

    % Quantification Vc -> uint16
    vc_q_double = round(double(vc_scalar) / double(vc_lsb));

    if vc_q_double < 0
        vc_q_double = 0;
    elseif vc_q_double > 65535
        vc_q_double = 65535;
    end

    vc_q = uint16(vc_q_double);

    % Quantification Iarm -> int16
    i_q_double = round(double(iarm_scalar) / double(i_lsb));

    if i_q_double < -32768
        i_q_double = -32768;
    elseif i_q_double > 32767
        i_q_double = 32767;
    end

    i_q = int16(i_q_double);

    % Conversion int16 -> uint16 sans typecast
    if i_q < int16(0)
        i_u16 = uint16(double(i_q) + 65536);
    else
        i_u16 = uint16(i_q);
    end

    frame = uint64(0);

    if valid
        frame = bitor(frame, bitshift(uint64(1), 41));
    end

    if current_present
        frame = bitor(frame, bitshift(uint64(1), 40));
    end

    frame = bitor(frame, bitshift(uint64(id_scalar), 32));
    frame = bitor(frame, bitshift(uint64(vc_q), 16));
    frame = bitor(frame, uint64(i_u16));
end

end

== matlab function MMC_phase_discentralized_HAAS_20260927/ /Subsystem/Subsystem1/Hardware M1/Power losses branch 1/Branch DT loss ==
  data: twist_FET_Pdt output; ILow input
function twist_FET_Pdt = powerLossesDeadTime(ILow)
    %Twist gate power losses
    twist_freq_switching = 200e3;
    twist_FET_Vf = 1.2;
    twist_FET_tDr = 10e-9;
    twist_FET_tDf = 0;

    twist_FET_Pdt = twist_FET_Vf*ILow*(twist_FET_tDr+twist_FET_tDf)*twist_freq_switching;
end
